simulink library "lib_IC_VSM"  (R2026a)
settings: Solver=VariableStepAuto
undefined symbols (not defined in the file): block_buses, block_DC_buses, block_DC_toM, block_idx, block_toM, buses_lf, DC, dparams, fb, fref, iC, inv2Hv, invL, iR, iTf, omegab, op_intconv_VSM
libraries: sl_discontinuities x1
(part 1 of 3)
settings Model: Creator=atomas  LastModifiedBy=atomas

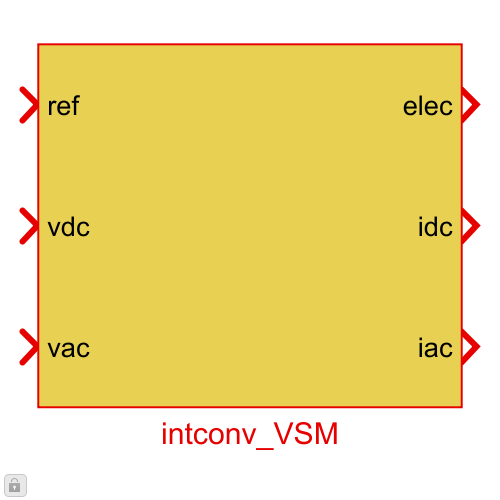
[thumbnail: Simulink's stored preview of the top-level diagram]
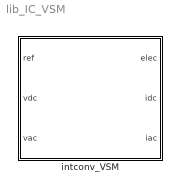
== system lib_IC_VSM ==
  intconv_VSM : Subsystem  mask(VCVSC){dynamic_VCC=Dynamic with P limitation, Lf=0.1, Rf=0.01, Rcf=1000000, Cfi=0.1, Kint=1, Tint=0.1, Bint=1, Kext=1, Bext=1, Text=0.1, Fi=1, Hv=3, Dv=0, Rv=0.05, nq=0.05, VI_L=0, VI_R=0, WOF_Tf=0, L_out=0.1, R_out=0.01, Tf=0.01, Kp_AC=0, Kd_AC=0, N_dc=100, Kp_theta=0, Kp_w=0, Ki_w=0, k_p_swing=1}
      mask prompts: dynamic_VCC "Dynamic behavior"; Lf "Filter inductance (pu)"; Rf "Filter resistance (pu)"; Rcf "Parallel resistance to C (pu)"; Cfi "Filter capacitance (pu)"; Fi "Current feedfordward gain"; Hv "Inertia"; Dv "Damping"; Rv "Droop Rv"; nq "Droop nq"; VI_L "Inductance (pu)"; VI_R "Resistance (pu)"; WOF_Tf "WOF time constant (s)"; L_out "Output inductance (p.u.)"; R_out "Output resistance (p.u.)"; Tf "Power filter time constant Tf (s):"; Kp_AC "DC-voltage proportional gain Kp_AC (pu):"; Kd_AC "DC-voltage derivative gain Kd_AC (pu*s):"; N_dc "DC-voltage derivative filter coefficient N_dc (rad/s):"; Kp_theta "ATM angle feed-forward gain Kp_theta (rad/pu):"; Kp_w "ATM frequency proportional gain Kp_w (pu/pu):"; Ki_w "ATM frequency integral gain Ki_w (pu/(pu*s)):"; k_p_swing "Swing equation DC-power coupling factor k_p_swing:"
      mask help: Grid-forming converter. VCC are the voltage and current controllers. Dynamic behavior includes the PI controllers, decoupling, current feedfordward and LC output filter. Static behavior consists of setting the reference voltage directly in the output. PC is the power controller including the droop control and low-pass filters for the power measurements.
      mask init:
      | [block_DC_buses, block_buses, block_DC_toM, block_toM, dparams, block_fref, block_idx, vcc_mode, use_wof_dc, use_kiw, use_Hv, inv2Hv] = mask_init_intconv_VSM(gcb, dynamic_VCC, Kd_AC, Ki_w, Hv);
      mask Help: web('Documentation/VCVSC.html')
      mask TypeOptions dynamic_VCC: Dynamic with limitation | Dynamic with P limitation | Dynamic | Static | Dynamic VC and static CC
      mask TypeOptions VI_L: VI/L
      mask TypeOptions VI_R: VI/R
      mask TypeOptions WOF_Tf: VI/Tf
      mask DialogControl Container8 Prompt: Parameters
      mask DialogControl VCC Prompt: VCC
      mask DialogControl PC Prompt: PC
      mask DialogControl VI Prompt: VI
      mask DialogControl Container9 Prompt: Others

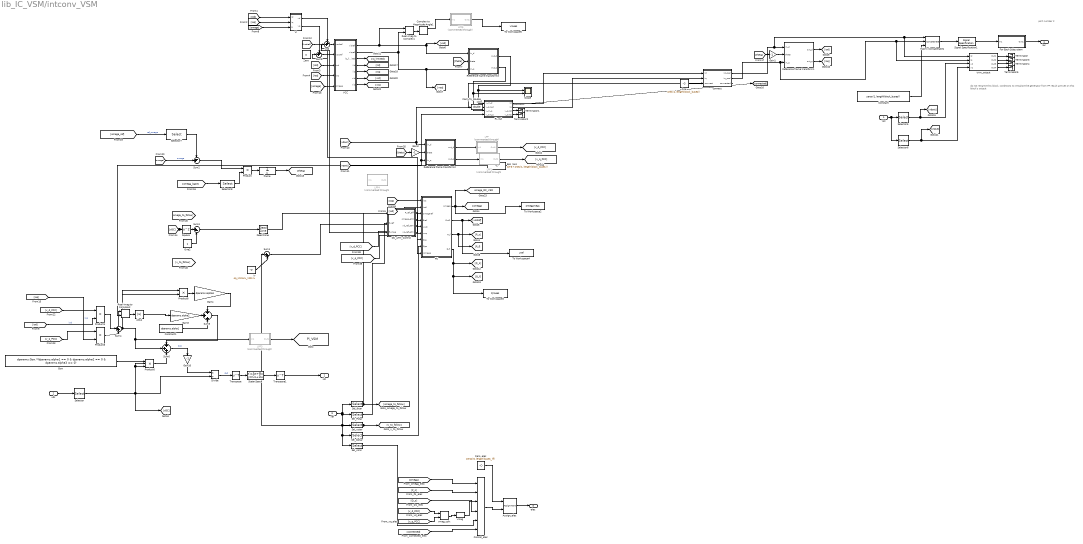
== system lib_IC_VSM/intconv_VSM ==
  note: do not rename this block, conditions to initialise the generator from PF result are set on this block's output
  note: port number 2
  vac : Inport
  vdc : Inport  Port=2
  ref : Inport  Port=3
  Abs4 : Abs  SaturateOnIntegerOverflow=off
  Assign_elec : Assignment  NumberOfDimensions=2  DiagnosticForDimensions=Warning  IndexOptions=Assign all,Index vector (dialog)  Indices=1,block_idx  OutputSizes=1
  Cast_To_Double_conn : DataTypeConversion  OutDataTypeStr=double
  Complex to Magnitude-Angle1 : ComplexToMagnitudeAngle
  Concat_elec : Concatenate  NumInputs=6  Mode=Multidimensional array
  Constant : Constant  Value=zeros(1, length(block_buses))  VectorParams1D=off
  Constant1 : Constant  Value=dparams.alpha1  VectorParams1D=off
  DC_ATM_Control : Subsystem
  Dead Zone : DeadZone  LowerValue=-0.2  UpperValue=0.2
  Divide : Product  Inputs=*/
  Eps_loss : Constant  Value=1e-6 * ones(1, length(block_buses))  VectorParams1D=off
  For Each Subsystem : Subsystem  TreatAsAtomicUnit=on
  Gain1 : Gain  Gain=-1
  Gain10 : Gain  Gain=-1
  Gain2 : Gain  Gain=-1
  Gain3 : Gain  Gain=dparams.alpha2
  Gain4 : Gain  Gain=dparams.alpha3
  Gsw : Constant  Value=dparams.Gsw.*(dparams.alpha1 == 0 & dparams.alpha2 == 0 & dparams.alpha3 == 0)  VectorParams1D=off
  LPF : Subsystem  Commented=through
  LPF1 : Subsystem  Commented=through
  LPF3 : Subsystem  Commented=through
  LPF4 : Subsystem  Commented=through
  LPF5 : Subsystem  Commented=through
  Matrix Concatenate1 : Concatenate  NumInputs=3  Mode=Multidimensional array
  One : Constant  Value=ones(1, length(block_buses))  VectorParams1D=off  OutDataTypeStr=Inherit: Inherit via back propagation
  One2 : Constant  OutDataTypeStr=Inherit: Inherit via back propagation
  PC : Subsystem  mask(PC_VCVSC){Tf=Tf, mp=0.01, nq=nq}
      mask prompts: Tf "Low-pass filter time constant (s)"; mp "Droop coefficient mp"; nq "Droop coefficient nq"
      mask help: Power controller of a grid-forming converter, including the droop control and low-pass filters for the power measurements.
      mask init:
      | [iTf, use_Tf] = mask_init_opt_filter(Tf);
  Product{,4..5,8} (4 alike) : Product
  Product6 : Product  Inputs=3
  RL out : Subsystem  Variant=on  mask{dynamic=Dynamic, R=dparams.Rf, L=dparams.Lf, fbase=50}
      mask prompts: dynamic "Dynamic behavior"; R "Series resistance (p.u.)"; L "Inductance (p.u.)"; fbase "Base frequency (Hz)"
      mask init:
      | [invL, omegab, rl_mode] = mask_init_RL(dynamic, L, fbase);
      mask TypeOptions dynamic: Static | Dynamic | Static omega
  Real-Imag to Complex1 : RealImagToComplex
  Real-Imag to Complex2 : RealImagToComplex
  Reference frame transform1 : Subsystem
  Reference frame transform2 : Subsystem
  Reference frame transform3 : Subsystem
  Scope : Scope  NumInputPorts=2
      settings: ActiveDisplayYMinimum=0.95813  ActiveDisplayYMaximum=1.0211
  Sel_Pstar : Selector  NumberOfDimensions=2  InputPortWidth=3  IndexOptions=Index vector (dialog),Index vector (dialog)  Indices=2,block_idx  OutputSizes=1
  Sel_Qstar : Selector  NumberOfDimensions=2  InputPortWidth=3  IndexOptions=Index vector (dialog),Index vector (dialog)  Indices=4,block_idx  OutputSizes=1
  Sel_conn : Selector  NumberOfDimensions=2  InputPortWidth=3  IndexOptions=Index vector (dialog),Index vector (dialog)  Indices=5,block_idx  OutputSizes=1
  Sel_fstar : Selector  NumberOfDimensions=2  InputPortWidth=3  IndexOptions=Index vector (dialog),Index vector (dialog)  Indices=1,block_idx  OutputSizes=1
  Sel_vstar : Selector  NumberOfDimensions=2  InputPortWidth=3  IndexOptions=Index vector (dialog),Index vector (dialog)  Indices=3,block_idx  OutputSizes=1
  Selector : Selector  InputPortWidth=DC.Nbuses  IndexOptions=Index vector (dialog)  Indices=block_DC_buses  OutputSizes=1
  Selector5 : Selector  NumberOfDimensions=2  InputPortWidth=3  IndexOptions=Index vector (dialog),Index vector (dialog)  Indices=1,block_buses  OutputSizes=1,1
  Selector6 : Selector  NumberOfDimensions=2  InputPortWidth=3  IndexOptions=Index vector (dialog),Index vector (dialog)  Indices=2,block_buses  OutputSizes=1,1
  Selector7 : Selector  InputPortWidth=length(fref.ref_units)  IndexOptions=Index vector (dialog)  Indices=block_fref  OutputSizes=1
  Selector8 : Selector  InputPortWidth=length(fref.ref_units)  IndexOptions=Index vector (dialog)  Indices=block_fref  OutputSizes=1
  Signal Specification1 : SignalSpecification  Dimensions=[3 length(block_buses)]
  Square : Math  Operator=square
  State-Space : StateSpace  A=[]  B=[]  C=[]  D=block_DC_toM  InitialCondition=0  ParameterTunability=Optimized
  Sum1 : Sum  Inputs=|++
  Sum2 : Sum  Inputs=-+|
  Sum3 : Sum  Inputs=|+-
  Sum4 : Sum  Inputs=|++
  Sum5 : Sum  Inputs=+|+|+
  Sum6 : Sum  Inputs=+|+|+
  Sum8 : Sum  Inputs=++|
  Terminator{,1..5} (6 alike) : Terminator
  To Workspace2 : ToWorkspace  VariableName=omegameas  SaveFormat=Timeseries  SampleTime=-1
  To Workspace3 : ToWorkspace  VariableName=Qmeas  SaveFormat=Timeseries  SampleTime=-1
  To Workspace4 : ToWorkspace  VariableName=vref  SaveFormat=Timeseries  SampleTime=-1
  To Workspace5 : ToWorkspace  VariableName=vmeas  SaveFormat=Timeseries  SampleTime=-1
  Transpose : Math  Operator=transpose
  Transpose1 : Math  Operator=transpose
  VCC : Subsystem  Variant=on
  VI : Subsystem  mask{L=VI_L, R=VI_R, Tf=WOF_Tf}
      mask prompts: L "Inductance (pu)"; R "Resistance (pu)"; Tf "WOF time constant (s)"
      mask init:
      | [iTf, use_Tf] = mask_init_opt_filter(Tf);
  Zero : Constant  Value=0  OutDataTypeStr=Inherit: Inherit via back propagation
  Zero_elec : Constant  Value=zeros(6, length(buses_lf))
  connect : Subsystem
  frame : Integrator  InitialCondition=op_intconv_VSM.frame  IgnoreLimit=on
  iv : Constant  Value=op_intconv_VSM.iv  VectorParams1D=off
  trim_output : Subsystem
  vmag : ComplexToMagnitudeAngle  Output=Magnitude
  vmag_cplx : RealImagToComplex
  vod : Sum  Inputs=++|
  iac : Outport
  idc : Outport  Port=2
  elec : Outport  Port=3
  tag scope: Pi_VSM=global, omega_DC_VSM=global
  wires:
  Sum8/1 -> VCC/2(voqref)
  vod/1 -> VCC/1(vodref)
  [omega] -> VI/3(omega)
  [ioq] -> VI/2(iq)
  [iod] -> VI/1(id)
  Gain2/1 -> Reference frame transform2/2(theta)
  [theta] -> Gain2/1
  PC/4(Q_f) -> [Q_s], To Workspace3/1, [Q_f]
  PC/3(P_f) -> [P_s], [P_f]
  [omega] -> Sum2/2  "omega"
  [omega_ref] -> Selector7/1  "ref_omega"
  RL out/1(id) -> connect/1(id)
  [theta] -> Gain1/1
  Gain1/1 -> Reference frame transform1/2(theta)
  [ioq] -> VCC/4(ioq)
  [iod] -> VCC/3(iod)
  [omega] -> VCC/5(omega)
  [theta] -> Reference frame transform3/2(theta)
  PC/1(omega) -> To Workspace2/1, [omega_DC_VSM], [omega]
  PC/2(Out2) -> To Workspace4/1, [vodref]
  [iod] -> PC/2(iodi)
  [ioq] -> PC/1(ioq)
  Reference frame transform1/2(out_q) -> [ioq]
  Reference frame transform3/1(out_d) -> RL out/1(v_in_d), Scope/1
  Reference frame transform3/2(out_q) -> RL out/3(v_in_q), Scope/2
  RL out/2(iq) -> connect/2(iq)
  Reference frame transform1/1(out_d) -> [iod]
  VI/1(vd) -> vod/1
  VI/2(vq) -> Sum8/1
  connect/1(id_real) -> trim_output/1(id), Matrix Concatenate1/1, Reference frame transform1/1(in_d)
  connect/2(iq_real) -> trim_output/2(iq), Matrix Concatenate1/2, Reference frame transform1/3(in_q)
  RL out/3(v_outd) -> Terminator1/1
  RL out/4(v_outq) -> Terminator2/1
  Reference frame transform2/1(out_d) -> LPF/1(In1)
  Reference frame transform2/2(out_q) -> LPF1/1(In1)
  [vqout] -> Reference frame transform2/3(in_q), RL out/4(v_out_q)
  LPF/1(Out1) -> [v_d_PCC]
  LPF1/1(Out1) -> [v_q_PCC]
  [vdout] -> RL out/2(v_out_d), Reference frame transform2/1(in_d)
  Matrix Concatenate1/1 -> Signal Specification1/1
  Constant/1 -> Matrix Concatenate1/3
  For Each Subsystem/1(Out1) -> iac/1
  Signal Specification1/1 -> For Each Subsystem/1(In1)
  [v_d_PCC] -> PC/5(vodi)
  [v_q_PCC] -> PC/6(voq)
  trim_output/1(Out1) -> Terminator/1
  trim_output/2(Out2) -> Terminator3/1
  trim_output/3(Out3) -> Terminator4/1
  trim_output/4(Out4) -> Terminator5/1
  vac/1 -> Selector6/1, Selector5/1
  Selector6/1 -> [vqout], trim_output/4(vq)
  Selector5/1 -> [vdout], trim_output/3(vd)
  VCC/1(vidref) -> Real-Imag to Complex1/1, [vod], Reference frame transform3/1(in_d)
  VCC/2(viqref) -> [voq], Reference frame transform3/3(in_q), Real-Imag to Complex1/2
  One/1 -> connect/3(connect)
  Sum1/1 -> PC/4(Eref)
  vdc/1 -> Selector/1
  Transpose/1 -> State-Space/1
  Divide/1 -> Transpose/1  "iDC"
  Abs4/1 -> Gain3/1
  Transpose1/1 -> idc/1
  Product5/1 -> Sum4/2
  Product6/1 -> Sum6/3
  Sum4/1 -> LPF3/1(In1), Sum6/2, Product8/1, Product8/2, Real-Imag to Complex2/1
  Sum5/1 -> Sum6/1
  State-Space/1 -> Transpose1/1
  Gain4/1 -> Sum5/1
  Gsw/1 -> Product6/1
  Real-Imag to Complex2/1 -> Abs4/1
  Constant1/1 -> Sum5/3
  Product4/1 -> Sum4/1
  Sum6/1 -> Gain10/1  "Pdc"
  Gain3/1 -> Sum5/2
  Gain10/1 -> Divide/1
  Product8/1 -> Gain4/1
  [v_q_PCC] -> Product5/1
  Selector/1 -> Product6/3, Product6/2, [vDC], Divide/2
  [ioq] -> Product5/2  "ioq"
  [v_d_PCC] -> Product4/1
  [iod] -> Product4/2  "iod"
  Product/1 -> frame/1
  VCC/3(iq_limited) -> [iq_limited]
  VCC/4(iid) -> [iid]
  VCC/5(iiq) -> [iiq]
  VCC/6(vid) -> [vid]
  VCC/7(viq) -> [viq]
  [vDC] -> Square/1, DC_ATM_Control/1(v_dc)
  Square/1 -> Sum3/1
  One2/1 -> Sum3/2
  frame/1 -> [theta]
  Sum3/1 -> Dead Zone/1
  LPF3/1(Out1) -> [Pi_VSM]
  Real-Imag to Complex1/1 -> Complex to Magnitude-Angle1/1
  Complex to Magnitude-Angle1/1 -> LPF5/1(In1)
  LPF5/1(Out1) -> To Workspace5/1
  Selector8/1 -> Product/2
  [omega_base] -> Selector8/1
  Sum2/1 -> Product/1
  Selector7/1 -> Sum2/1
  ref/1 -> Sel_Qstar/1, Sel_conn/1, Sel_vstar/1, Sel_Pstar/1, Sel_fstar/1
  Sel_fstar/1 -> [omega_to_follow], PC/3(omegaref)
  Sel_vstar/1 -> [v_to_follow], Sum1/1
  Sel_Qstar/1 -> PC/8(Qsp)
  [v_d_PCC] -> vmag_cplx/1
  [v_q_PCC] -> vmag_cplx/2
  vmag_cplx/1 -> vmag/1
  [omega] -> Concat_elec/1
  [P_s] -> Concat_elec/2
  vmag/1 -> Concat_elec/3
  [Q_s] -> Concat_elec/4
  Sel_conn/1 -> Concat_elec/5
  [connected] -> Concat_elec/6
  Zero_elec/1 -> Assign_elec/1
  Concat_elec/1 -> Assign_elec/2
  Assign_elec/1 -> elec/1
  Sel_Pstar/1 -> DC_ATM_Control/2(P_ref)
  [vodref] -> DC_ATM_Control/3(E_mag)
  DC_ATM_Control/1(P_ref_eff) -> PC/7(Psp)
  DC_ATM_Control/2(omega_atm) -> PC/9(iomega)
  DC_ATM_Control/3(vd_ref_atm) -> vod/2
  DC_ATM_Control/4(vq_ref_atm) -> Sum8/2
  iv/1 -> Sum1/2
  Eps_loss/1 -> Real-Imag to Complex2/2
  connect/3(connected) -> Cast_To_Double_conn/1
  Cast_To_Double_conn/1 -> [connected]

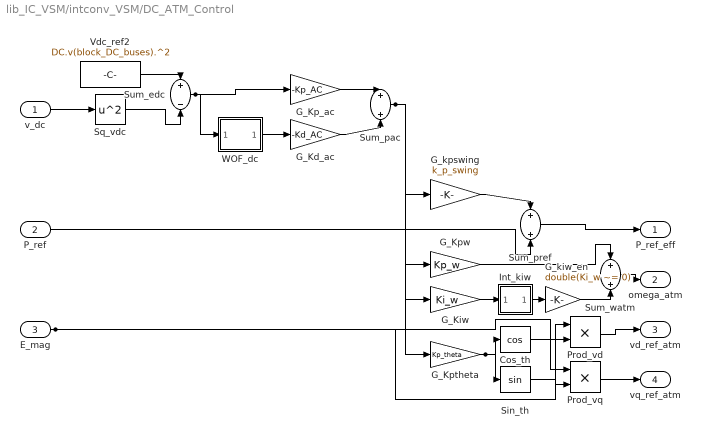
== system lib_IC_VSM/intconv_VSM/DC_ATM_Control ==
  v_dc : Inport
  P_ref : Inport  Port=2
  E_mag : Inport  Port=3
  Cos_th : Trigonometry  Operator=cos
  G_Kd_ac : Gain  Gain=-Kd_AC
  G_Kiw : Gain  Gain=Ki_w
  G_Kp_ac : Gain  Gain=-Kp_AC
  G_Kptheta : Gain  Gain=Kp_theta
  G_Kpw : Gain  Gain=Kp_w
  G_kiw_en : Gain  Gain=double(Ki_w ~= 0)
  G_kpswing : Gain  Gain=k_p_swing
  Int_kiw : Subsystem  Variant=on
  Prod_vd : Product  Inputs=**
  Prod_vq : Product  Inputs=**
  Sin_th : Trigonometry
  Sq_vdc : Math  Operator=square
  Sum_edc : Sum  Inputs=+-
  Sum_pac : Sum
  Sum_pref : Sum
  Sum_watm : Sum
  Vdc_ref2 : Constant  Value=DC.v(block_DC_buses).^2
  WOF_dc : Subsystem  Variant=on
  P_ref_eff : Outport
  omega_atm : Outport  Port=2
  vd_ref_atm : Outport  Port=3
  vq_ref_atm : Outport  Port=4
  wires:
  Int_kiw/1(Out1) -> G_kiw_en/1
  G_Kiw/1 -> Int_kiw/1(In1)
  WOF_dc/1(Out1) -> G_Kd_ac/1
  Sum_edc/1 -> WOF_dc/1(In1), G_Kp_ac/1
  v_dc/1 -> Sq_vdc/1
  Vdc_ref2/1 -> Sum_edc/1
  Sq_vdc/1 -> Sum_edc/2
  G_Kp_ac/1 -> Sum_pac/1
  G_Kd_ac/1 -> Sum_pac/2
  Sum_pac/1 -> G_kpswing/1, G_Kpw/1, G_Kiw/1, G_Kptheta/1
  G_kpswing/1 -> Sum_pref/1
  P_ref/1 -> Sum_pref/2
  Sum_pref/1 -> P_ref_eff/1
  G_Kpw/1 -> Sum_watm/1
  G_kiw_en/1 -> Sum_watm/2
  Sum_watm/1 -> omega_atm/1
  G_Kptheta/1 -> Cos_th/1, Sin_th/1
  E_mag/1 -> Prod_vd/1, Prod_vq/1
  Cos_th/1 -> Prod_vd/2
  Sin_th/1 -> Prod_vq/2
  Prod_vd/1 -> vd_ref_atm/1
  Prod_vq/1 -> vq_ref_atm/1

== system lib_IC_VSM/intconv_VSM/For Each Subsystem ==
  In1 : Inport  Partition=on  PartitionDimension=1  PartitionWidth=1  PartitionOffset=0
  For Each : ForEach  DisableCoverage=on
  State-Space : StateSpace  A=[]  B=[]  C=[]  D=block_toM  InitialCondition=0  ParameterTunability=Optimized
  Transpose : Math  Operator=transpose
  Transpose1 : Math  Operator=transpose
  Out1 : Outport  ConcatenationDimension=1
  wires:
  State-Space/1 -> Transpose1/1
  Transpose/1 -> State-Space/1
  Transpose1/1 -> Out1/1
  In1/1 -> Transpose/1

== system lib_IC_VSM/intconv_VSM/LPF ==
  In1 : Inport
  Gain : Gain  Gain=1e2
  I : Integrator  InitialCondition=op_intconv_VSM.LPF_I
  Sum4 : Sum  Inputs=|+-
  Out1 : Outport
  wires:
  Gain/1 -> I/1
  Sum4/1 -> Gain/1
  In1/1 -> Sum4/1
  I/1 -> Out1/1, Sum4/2

== system lib_IC_VSM/intconv_VSM/LPF1 ==
  In1 : Inport
  Gain : Gain  Gain=1e2
  I : Integrator  InitialCondition=op_intconv_VSM.LPF1_I
  Sum4 : Sum  Inputs=|+-
  Out1 : Outport
  wires:
  I/1 -> Sum4/2, Out1/1
  In1/1 -> Sum4/1
  Sum4/1 -> Gain/1
  Gain/1 -> I/1

== system lib_IC_VSM/intconv_VSM/LPF3 ==
  In1 : Inport
  Gain : Gain  Gain=1000
  I : Integrator  InitialCondition=op_intconv_VSM.LPF3_I
  Sum4 : Sum  Inputs=|+-
  Out1 : Outport
  wires:
  Gain/1 -> I/1
  Sum4/1 -> Gain/1
  In1/1 -> Sum4/1
  I/1 -> Out1/1, Sum4/2

== system lib_IC_VSM/intconv_VSM/LPF4 ==
  In1 : Inport
  Gain : Gain  Gain=1e2
  I : Integrator  InitialCondition=op_intconv_VSM.LPF4_I
  Sum4 : Sum  Inputs=|+-
  Out1 : Outport
  wires:
  Gain/1 -> I/1
  Sum4/1 -> Gain/1
  In1/1 -> Sum4/1
  I/1 -> Out1/1, Sum4/2

== system lib_IC_VSM/intconv_VSM/LPF5 ==
  In1 : Inport
  Gain : Gain  Gain=1e4
  I : Integrator  InitialConditionSource=external  InitialCondition=op_intconv_VSM.LPF5_I
  Sum4 : Sum  Inputs=|+-
  Out1 : Outport
  wires:
  Gain/1 -> I/1
  Sum4/1 -> Gain/1
  In1/1 -> I/2, Sum4/1
  I/1 -> Out1/1, Sum4/2

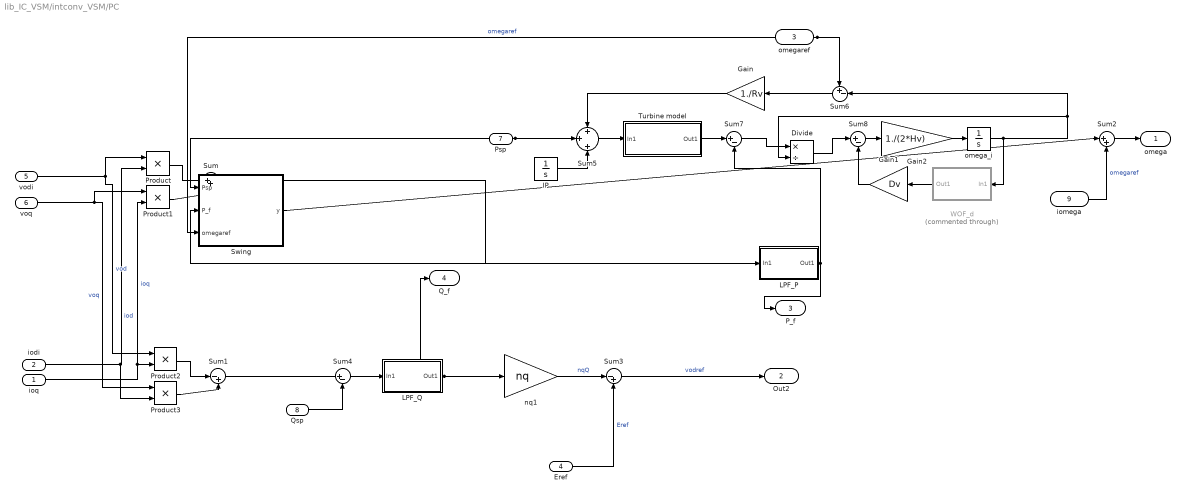
== system lib_IC_VSM/intconv_VSM/PC ==
  ioq : Inport
  iodi : Inport  Port=2
  omegaref : Inport  Port=3
  Eref : Inport  Port=4
  vodi : Inport  Port=5
  voq : Inport  Port=6
  Psp : Inport  Port=7
  Qsp : Inport  Port=8
  iomega : Inport  Port=9
  Divide : Product  Inputs=*/
  Gain : Gain  Gain=1./Rv
  Gain1 : Gain  Gain=Dv
  Gain2 : Gain  Gain=1./(2*Hv)
  IP : Integrator  InitialCondition=op_intconv_VSM.PC_IP
  LPF_P : Subsystem  Variant=on
  LPF_Q : Subsystem  Variant=on
  Product{,1..3} (4 alike) : Product
  Sum : Sum  Inputs=|++
  Sum1 : Sum  Inputs=|-+
  Sum2 : Sum  Inputs=|++
  Sum3 : Sum  Inputs=|-+
  Sum4 : Sum  Inputs=|+-
  Sum5 : Sum  Inputs=+|+|+
  Sum6 : Sum  Inputs=+-|
  Sum7 : Sum  Inputs=|+-
  Sum8 : Sum  Inputs=|+-
  Swing : Subsystem  Variant=on
  Turbine model : Subsystem
  WOF_d : Subsystem  Commented=through
  nq1 : Gain  Gain=nq
  omega_i : Integrator  InitialCondition=op_intconv_VSM.PC_omega_i
  omega : Outport
  Out2 : Outport  Port=2
  P_f : Outport  Port=3
  Q_f : Outport  Port=4
  wires:
  LPF_P/1(Out1) -> Sum7/2, P_f/1, Swing/2(P_f)
  Sum/1 -> LPF_P/1(In1)
  vodi/1 -> Product2/1, Product/1  "vod"
  Product/1 -> Sum/1
  Product1/1 -> Sum/2
  Product2/1 -> Sum1/1
  Product3/1 -> Sum1/2
  nq1/1 -> Sum3/1  "nqQ"
  Eref/1 -> Sum3/2  "Eref"
  voq/1 -> Product1/1, Product3/1  "voq"
  iodi/1 -> Product3/2, Product/2  "iod"
  ioq/1 -> Product2/2, Product1/2  "ioq"
  Qsp/1 -> Sum4/2
  Sum3/1 -> Out2/1  "vodref"
  Gain2/1 -> omega_i/1
  Sum6/1 -> Gain/1
  omega_i/1 -> WOF_d/1(In1), Sum6/2, Divide/2
  Gain/1 -> Sum5/1
  WOF_d/1(Out1) -> Gain1/1
  Turbine model/1(Out1) -> Sum7/1
  Gain1/1 -> Sum8/2
  Divide/1 -> Sum8/1
  Psp/1 -> Sum5/2, Swing/1(Psp)
  Sum5/1 -> Turbine model/1(In1)
  Sum7/1 -> Divide/1
  Sum8/1 -> Gain2/1
  IP/1 -> Sum5/3
  omegaref/1 -> Sum6/1, Swing/3(omegaref)  "omegaref"
  Sum2/1 -> omega/1
  iomega/1 -> Sum2/2  "omegaref"
  Sum1/1 -> LPF_Q/1(In1)
  LPF_Q/1(Out1) -> Q_f/1, Sum4/1
  Sum4/1 -> nq1/1
  Swing/1(y) -> Sum2/1

== system lib_IC_VSM/intconv_VSM/RL out ==
  note: 1) Add Subsystem or Model blocks as valid variant choices.
      | 2) You cannot connect blocks at this level. At simulation, connectivity is automatically
      | determined, based on the active variant and port name matching.
  v_in_d : Inport
  v_out_d : Inport  Port=2
  v_in_q : Inport  Port=3
  v_out_q : Inport  Port=4
  dynamic : Subsystem  VariantControl=rl_mode == 1
  static : Subsystem  VariantControl=rl_mode == 2
  static_omega : Subsystem  VariantControl=(default)
  id : Outport
  iq : Outport  Port=2
  v_outd : Outport  Port=3
  v_outq : Outport  Port=4

== system lib_IC_VSM/intconv_VSM/Reference frame transform1 ==
  in_d : Inport
  theta : Inport  Port=2
  in_q : Inport  Port=3
  Complex to Real-Imag : ComplexToRealImag
  Cos : Trigonometry  SCDEnableBlockLinearizationSpecification=on  Operator=cos
  Product : Product
  Real-Imag to Complex : RealImagToComplex
  Real-Imag to Complex1 : RealImagToComplex
  Sin : Trigonometry  SCDEnableBlockLinearizationSpecification=on
  out_d : Outport
  out_q : Outport  Port=2
  wires:
  Complex to Real-Imag/2 -> out_q/1
  Real-Imag to Complex1/1 -> Product/1
  Real-Imag to Complex/1 -> Product/2
  Product/1 -> Complex to Real-Imag/1
  theta/1 -> Sin/1, Cos/1
  Cos/1 -> Real-Imag to Complex1/1
  Sin/1 -> Real-Imag to Complex1/2
  Complex to Real-Imag/1 -> out_d/1
  in_q/1 -> Real-Imag to Complex/2
  in_d/1 -> Real-Imag to Complex/1

== system lib_IC_VSM/intconv_VSM/Reference frame transform2 ==
  in_d : Inport
  theta : Inport  Port=2
  in_q : Inport  Port=3
  Complex to Real-Imag : ComplexToRealImag
  Cos : Trigonometry  SCDEnableBlockLinearizationSpecification=on  Operator=cos
  Product : Product
  Real-Imag to Complex : RealImagToComplex
  Real-Imag to Complex1 : RealImagToComplex
  Sin : Trigonometry  SCDEnableBlockLinearizationSpecification=on
  out_d : Outport
  out_q : Outport  Port=2
  wires:
  in_d/1 -> Real-Imag to Complex/1
  in_q/1 -> Real-Imag to Complex/2
  Complex to Real-Imag/1 -> out_d/1
  Sin/1 -> Real-Imag to Complex1/2
  Cos/1 -> Real-Imag to Complex1/1
  theta/1 -> Cos/1, Sin/1
  Product/1 -> Complex to Real-Imag/1
  Real-Imag to Complex/1 -> Product/2
  Real-Imag to Complex1/1 -> Product/1
  Complex to Real-Imag/2 -> out_q/1

== system lib_IC_VSM/intconv_VSM/Reference frame transform3 ==
  in_d : Inport
  theta : Inport  Port=2
  in_q : Inport  Port=3
  Complex to Real-Imag : ComplexToRealImag
  Cos : Trigonometry  SCDEnableBlockLinearizationSpecification=on  Operator=cos
  Product : Product
  Real-Imag to Complex : RealImagToComplex
  Real-Imag to Complex1 : RealImagToComplex
  Sin : Trigonometry  SCDEnableBlockLinearizationSpecification=on
  out_d : Outport
  out_q : Outport  Port=2
  wires:
  Complex to Real-Imag/2 -> out_q/1
  Real-Imag to Complex1/1 -> Product/1
  Real-Imag to Complex/1 -> Product/2
  Product/1 -> Complex to Real-Imag/1
  theta/1 -> Cos/1, Sin/1
  Cos/1 -> Real-Imag to Complex1/1
  Sin/1 -> Real-Imag to Complex1/2
  Complex to Real-Imag/1 -> out_d/1
  in_q/1 -> Real-Imag to Complex/2
  in_d/1 -> Real-Imag to Complex/1

== system lib_IC_VSM/intconv_VSM/VCC ==
  note: 1) Add Subsystem or Model blocks as valid variant choices.
      | 2) You cannot connect blocks at this level. At simulation, connectivity is automatically
      | determined, based on the active variant and port name matching.
  vodref : Inport
  voqref : Inport  Port=2
  iod : Inport  Port=3
  ioq : Inport  Port=4
  omega : Inport  Port=5
  dynamic : Subsystem  VariantControl=vcc_mode == 1
  dynamic_VC : Subsystem  VariantControl=vcc_mode == 3
  dynamic_limiting : Subsystem  VariantControl=vcc_mode == 2
  dynamic_limiting_P : Subsystem  VariantControl=vcc_mode == 4
  static : Subsystem  VariantControl=(default)
  vidref : Outport
  viqref : Outport  Port=2
  iq_limited : Outport  Port=3
  iid : Outport  Port=4
  iiq : Outport  Port=5
  vid : Outport  Port=6
  viq : Outport  Port=7

== system lib_IC_VSM/intconv_VSM/VI ==
  id : Inport
  iq : Inport  Port=2
  omega : Inport  Port=3
  Gain : Gain  Gain=L
  Gain1 : Gain  Gain=R
  Gain2 : Gain  Gain=L
  Gain3 : Gain  Gain=R
  Product : Product
  Product1 : Product
  Sum : Sum  Inputs=-+|
  Sum1 : Sum  Inputs=|--
  WOF_d : Subsystem  Variant=on
  WOF_q : Subsystem  Variant=on
  vd : Outport
  vq : Outport  Port=2
  wires:
  WOF_q/1(Out1) -> Gain/1, Gain3/1
  iq/1 -> WOF_q/1(In1)
  WOF_d/1(Out1) -> Gain1/1, Gain2/1
  id/1 -> WOF_d/1(In1)
  Sum1/1 -> vq/1
  Sum/1 -> vd/1
  Gain3/1 -> Sum1/2
  Gain1/1 -> Sum/1
  Product1/1 -> Sum1/1
  Gain2/1 -> Product1/2
  Product/1 -> Sum/2
  omega/1 -> Product1/1, Product/2
  Gain/1 -> Product/1

== system lib_IC_VSM/intconv_VSM/connect ==
  id : Inport
  iq : Inport  Port=2
  connect : Inport  Port=3
  Switch : Switch  Criteria=u2 > Threshold  ZeroCross=off  SaturateOnIntegerOverflow=off  InputSameDT=off
  Switch1 : Switch  Criteria=u2 > Threshold  ZeroCross=off  SaturateOnIntegerOverflow=off  InputSameDT=off
  Zero1 : Constant  Value=0  VectorParams1D=off  OutDataTypeStr=Inherit: Inherit via back propagation
  Zero2 : Constant  Value=0  VectorParams1D=off  OutDataTypeStr=Inherit: Inherit via back propagation
  id_real : Outport
  iq_real : Outport  Port=2
  connected : Outport  Port=3  OutDataTypeStr=boolean
  wires:
  Switch/1 -> id_real/1
  Zero1/1 -> Switch/3
  id/1 -> Switch/1
  connect/1 -> connected/1, Switch1/2, Switch/2
  Switch1/1 -> iq_real/1
  iq/1 -> Switch1/1
  Zero2/1 -> Switch1/3

== system lib_IC_VSM/intconv_VSM/trim_output ==
  id : Inport
  iq : Inport  Port=2
  vd : Inport  Port=3
  vq : Inport  Port=4
  Out1 : Outport
  Out2 : Outport  Port=2
  Out3 : Outport  Port=3
  Out4 : Outport  Port=4
  wires:
  id/1 -> Out1/1
  vq/1 -> Out4/1
  vd/1 -> Out3/1
  iq/1 -> Out2/1

== system lib_IC_VSM/intconv_VSM/DC_ATM_Control/Int_kiw ==
  note: 1) Add Subsystem or Model blocks as valid variant choices.
      | 2) You cannot connect blocks at this level. At simulation, connectivity is automatically
      | determined, based on the active variant and port name matching.
  In1 : Inport
  Active : Subsystem  VariantControl=use_kiw == 1
  Bypass : Subsystem  VariantControl=(default)
  Out1 : Outport

== system lib_IC_VSM/intconv_VSM/DC_ATM_Control/WOF_dc ==
  note: 1) Add Subsystem or Model blocks as valid variant choices.
      | 2) You cannot connect blocks at this level. At simulation, connectivity is automatically
      | determined, based on the active variant and port name matching.
  In1 : Inport
  Active : Subsystem  VariantControl=use_wof_dc == 1
  Bypass : Subsystem  VariantControl=(default)
  Out1 : Outport

== system lib_IC_VSM/intconv_VSM/PC/LPF_P ==
  note: 1) Add Subsystem or Model blocks as valid variant choices.
      | 2) You cannot connect blocks at this level. At simulation, connectivity is automatically
      | determined, based on the active variant and port name matching.
  In1 : Inport
  Active : Subsystem  VariantControl=use_Tf == 1
  Bypass : Subsystem  VariantControl=(default)
  Out1 : Outport

== system lib_IC_VSM/intconv_VSM/PC/LPF_Q ==
  note: 1) Add Subsystem or Model blocks as valid variant choices.
      | 2) You cannot connect blocks at this level. At simulation, connectivity is automatically
      | determined, based on the active variant and port name matching.
  In1 : Inport
  Active : Subsystem  VariantControl=use_Tf == 1
  Bypass : Subsystem  VariantControl=(default)
  Out1 : Outport

== system lib_IC_VSM/intconv_VSM/PC/Swing ==
  note: 1) Add Subsystem or Model blocks as valid variant choices.
      | 2) You cannot connect blocks at this level. At simulation, connectivity is automatically
      | determined, based on the active variant and port name matching.
  Psp : Inport
  P_f : Inport  Port=2
  omegaref : Inport  Port=3
  Active : Subsystem  VariantControl=use_Hv == 1
  Droop : Subsystem  VariantControl=(default)
  y : Outport

== system lib_IC_VSM/intconv_VSM/PC/Turbine model ==
  In1 : Inport
  Out1 : Outport
  wires:
  In1/1 -> Out1/1

== system lib_IC_VSM/intconv_VSM/PC/WOF_d ==
  In1 : Inport
  Gain : Gain  Gain=10
  Gain1 : Gain  Gain=10
  I : Integrator  InitialConditionSource=external  InitialCondition=op_intconv_VSM.PC_WOF_d_I
  Sum : Sum  Inputs=+-|
  Sum4 : Sum  Inputs=|+-
  Out1 : Outport
  wires:
  Gain/1 -> I/1
  Sum4/1 -> Gain/1
  In1/1 -> I/2, Sum/1, Sum4/1
  I/1 -> Sum/2, Sum4/2
  Sum/1 -> Gain1/1
  Gain1/1 -> Out1/1

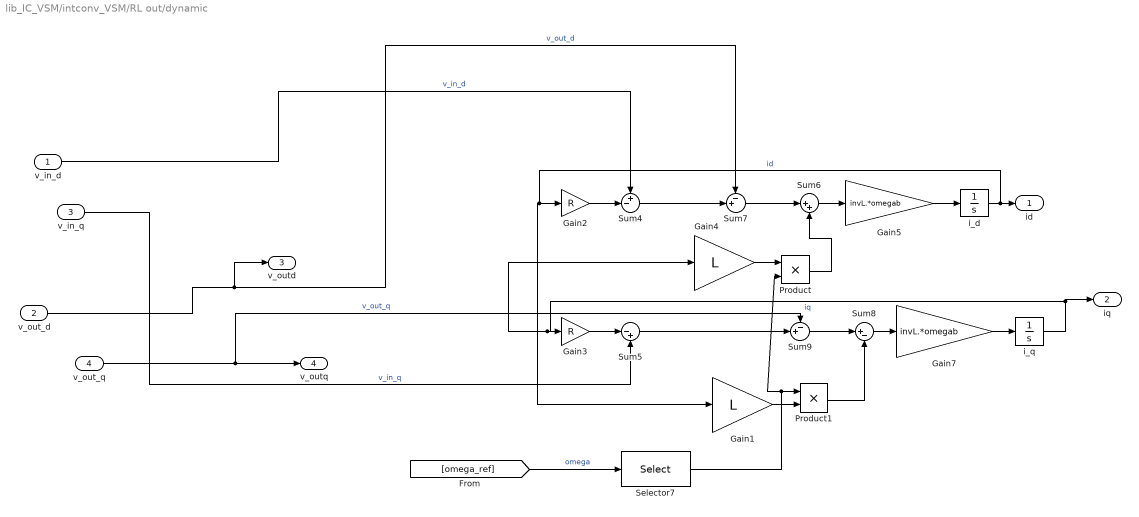
== system lib_IC_VSM/intconv_VSM/RL out/dynamic ==
  v_in_d : Inport
  v_out_d : Inport  Port=2
  v_in_q : Inport  Port=3
  v_out_q : Inport  Port=4
  Gain1 : Gain  Gain=L
  Gain2 : Gain  Gain=R
  Gain3 : Gain  Gain=R
  Gain4 : Gain  Gain=L
  Gain5 : Gain  Gain=invL.*omegab
  Gain7 : Gain  Gain=invL.*omegab
  Product : Product
  Product1 : Product
  Selector7 : Selector  InputPortWidth=length(fref.ref_units)  IndexOptions=Index vector (dialog)  Indices=block_fref  OutputSizes=1
  Sum4 : Sum  Inputs=+-|
  Sum5 : Sum  Inputs=|-+
  Sum6 : Sum  Inputs=|++
  Sum7 : Sum  Inputs=-+|
  Sum8 : Sum  Inputs=|+-
  Sum9 : Sum  Inputs=-+|
  i_d : Integrator  InitialCondition=op_intconv_VSM.RL_out_dynamic_i_d
  i_q : Integrator  InitialCondition=op_intconv_VSM.RL_out_dynamic_i_q
  id : Outport
  iq : Outport  Port=2
  v_outd : Outport  Port=3
  v_outq : Outport  Port=4
  wires:
  v_out_q/1 -> v_outq/1, Sum9/1  "v_out_q"
  v_out_d/1 -> v_outd/1, Sum7/1  "v_out_d"
  Sum9/1 -> Sum8/1
  Gain1/1 -> Product1/2
  i_q/1 -> iq/1, Gain4/1, Gain3/1  "iq"
  Gain7/1 -> i_q/1
  Sum5/1 -> Sum9/2
  Gain3/1 -> Sum5/1
  Sum7/1 -> Sum6/1
  Gain4/1 -> Product/1
  Product1/1 -> Sum8/2
  Sum4/1 -> Sum7/2
  Sum8/1 -> Gain7/1
  Product/1 -> Sum6/2
  Gain5/1 -> i_d/1
  [omega_ref] -> Selector7/1  "omega"
  Sum6/1 -> Gain5/1
  i_d/1 -> id/1, Gain1/1, Gain2/1  "id"
  Gain2/1 -> Sum4/2
  v_in_d/1 -> Sum4/1  "v_in_d"
  v_in_q/1 -> Sum5/2  "v_in_q"
  Selector7/1 -> Product/2, Product1/1

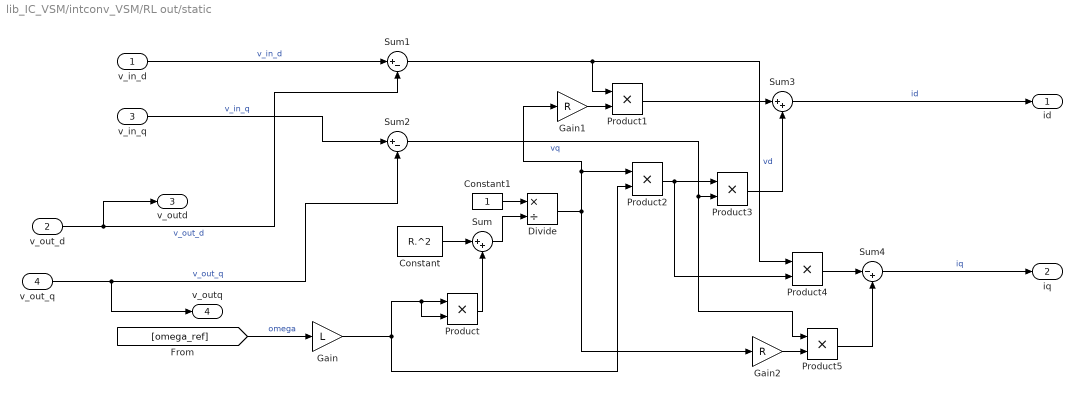
== system lib_IC_VSM/intconv_VSM/RL out/static ==
  v_in_d : Inport
  v_out_d : Inport  Port=2
  v_in_q : Inport  Port=3
  v_out_q : Inport  Port=4
  Constant : Constant  Value=R.^2
  Constant1 : Constant
  Divide : Product  Inputs=*/
  Gain : Gain  Gain=L
  Gain1 : Gain  Gain=R
  Gain2 : Gain  Gain=R
  Product{,1..5} (6 alike) : Product
  Sum : Sum  Inputs=|++
  Sum1 : Sum  Inputs=|+-
  Sum2 : Sum  Inputs=|+-
  Sum3 : Sum  Inputs=|++
  Sum4 : Sum  Inputs=|-+
  id : Outport
  iq : Outport  Port=2
  v_outd : Outport  Port=3
  v_outq : Outport  Port=4
  wires:
  [omega_ref] -> Gain/1  "omega"
  v_in_d/1 -> Sum1/1  "v_in_d"
  v_out_q/1 -> v_outq/1, Sum2/2  "v_out_q"
  Sum4/1 -> iq/1  "iq"
  Sum3/1 -> id/1  "id"
  Gain1/1 -> Product1/2
  Product2/1 -> Product4/2, Product3/1
  Product4/1 -> Sum4/1
  Divide/1 -> Gain2/1, Gain1/1, Product2/1
  Sum1/1 -> Product1/1, Product4/1  "vd"
  Product3/1 -> Sum3/2
  Constant1/1 -> Divide/1
  Gain/1 -> Product/2, Product/1, Product2/2
  Sum2/1 -> Product5/1, Product3/2  "vq"
  Constant/1 -> Sum/1
  Product5/1 -> Sum4/2
  Product1/1 -> Sum3/1
  Product/1 -> Sum/2
  Gain2/1 -> Product5/2
  Sum/1 -> Divide/2
  v_out_d/1 -> v_outd/1, Sum1/2  "v_out_d"
  v_in_q/1 -> Sum2/1  "v_in_q"

== system lib_IC_VSM/intconv_VSM/RL out/static_omega ==
  v_in_d : Inport
  v_out_d : Inport  Port=2
  v_in_q : Inport  Port=3
  v_out_q : Inport  Port=4
  Gain : Gain  Gain=1./(R.^2+L.^2)
  Gain2 : Gain  Gain=1./(R.^2+L.^2)
  Gain3 : Gain  Gain=R
  Gain4 : Gain  Gain=L
  Gain5 : Gain  Gain=L
  Gain6 : Gain  Gain=R
  Sum : Sum  Inputs=|++
  Sum1 : Sum  Inputs=|+-
  Sum2 : Sum  Inputs=|+-
  Sum3 : Sum  Inputs=|-+
  id : Outport
  iq : Outport  Port=2
  v_outd : Outport  Port=3
  v_outq : Outport  Port=4
  wires:
  v_in_q/1 -> Sum2/1  "v_in_q"
  v_in_d/1 -> Sum1/1  "v_in_d"
  v_out_q/1 -> v_outq/1, Sum2/2  "v_out_q"
  v_out_d/1 -> v_outd/1, Sum1/2  "v_out_d"
  Sum1/1 -> Gain/1  "vd"
  Sum2/1 -> Gain2/1  "vq"
  Gain/1 -> Gain5/1, Gain3/1
  Gain3/1 -> Sum/1
  Gain4/1 -> Sum/2
  Gain2/1 -> Gain6/1, Gain4/1
  Sum/1 -> id/1
  Gain5/1 -> Sum3/1
  Sum3/1 -> iq/1
  Gain6/1 -> Sum3/2

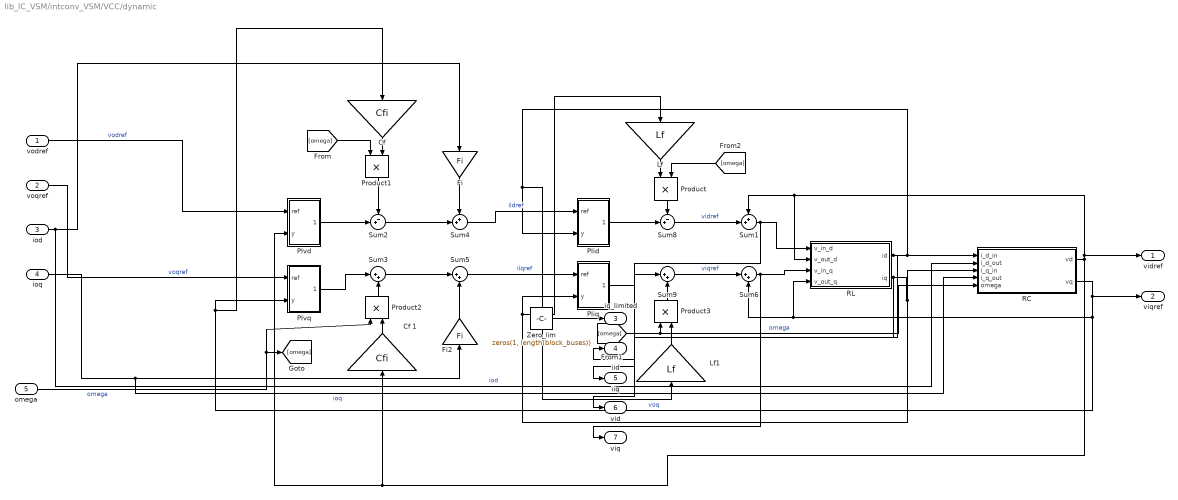
== system lib_IC_VSM/intconv_VSM/VCC/dynamic ==
  vodref : Inport
  voqref : Inport  Port=2
  iod : Inport  Port=3
  ioq : Inport  Port=4
  omega : Inport  Port=5
  Cf : Gain  Gain=Cfi
  Cf 1 : Gain  Gain=Cfi
  Fi : Gain  Gain=Fi
  Fi2 : Gain  Gain=Fi
  "Lf " : Gain  Gain=Lf
  Lf1 : Gain  Gain=Lf
  PIid : Subsystem
  PIiq : Subsystem
  PIvd : Subsystem
  PIvq : Subsystem
  Product{,1..3} (4 alike) : Product
  RC : Subsystem  Variant=on  mask{dynamic=Dynamic, R=Rcf, C=Cfi, fbase=50}
      mask prompts: dynamic "Dynamic behavior"; R "Parallel resistance (p.u.)"; C "Capacitance (p.u.)"; fbase "Base frequency (Hz)"
      mask init:
      | [iC, iR, omegab, rc_mode] = mask_init_RC(dynamic, R, C, fbase);
      mask TypeOptions dynamic: Dynamic | Static | Static omega
  RL : Subsystem  Variant=on  mask(Line){dynamic=Dynamic, R=Rf, L=Lf, fbase=fb}
      mask prompts: dynamic "Dynamic behavior"; R "Series resistance (p.u.)"; L "Inductance (p.u.)"; fbase "Base frequency (Hz)"
      mask init:
      | [invL, omegab, rl_mode] = mask_init_RL(dynamic, L, fbase);
      mask Help: web('Documentation/RL.html')
      mask TypeOptions dynamic: Static | Dynamic | Static omega
  Sum1 : Sum  Inputs=++|
  Sum2 : Sum  Inputs=-+|
  Sum{3,5..6,9} (4 alike) : Sum  Inputs=|++
  Sum4 : Sum  Inputs=++|
  Sum8 : Sum  Inputs=-+|
  Zero_lim : Constant  Value=zeros(1, length(block_buses))
  vidref : Outport
  viqref : Outport  Port=2
  iq_limited : Outport  Port=3
  iid : Outport  Port=4
  iiq : Outport  Port=5
  vid : Outport  Port=6
  viq : Outport  Port=7
  wires:
  Sum5/1 -> PIiq/1(ref)  "ilqref"
  Product/1 -> Sum8/1
  vodref/1 -> PIvd/1(ref)  "vodref"
  RC/2(vq) -> viqref/1, Sum6/2, RL/4(v_out_q), PIvq/2(y), Cf/1  "voq"
  [omega] -> Product/2
  Lf1/1 -> Product3/2
  Fi/1 -> Sum4/1
  voqref/1 -> PIvq/1(ref)  "voqref"
  Product3/1 -> Sum9/2
  Product2/1 -> Sum3/2
  Cf 1/1 -> Product2/2
  Cf/1 -> Product1/2
  Sum4/1 -> PIid/1(ref)  "ildref"
  Product1/1 -> Sum2/1
  iod/1 -> RC/2(i_d_out), Fi/1  "iod"
  Sum2/1 -> Sum4/2
  "Lf "/1 -> Product/1
  Sum3/1 -> Sum5/1
  [omega] -> RC/5(omega), Product3/1  "omega"
  ioq/1 -> RC/4(i_q_out), Fi2/1  "ioq"
  Fi2/1 -> Sum5/2
  PIvd/1(Out1) -> Sum2/2
  PIvq/1(Out1) -> Sum3/1
  PIid/1(Out1) -> Sum8/2
  PIiq/1(Out1) -> Sum9/1
  omega/1 -> Product2/1, [omega]  "omega"
  [omega] -> Product1/1
  RC/1(vd) -> vidref/1, Sum1/1, RL/2(v_out_d), PIvd/2(y), Cf 1/1
  RL/1(id) -> PIid/2(y), Lf1/1, RC/1(i_d_in), iid/1
  RL/2(iq) -> RC/3(i_q_in), PIiq/2(y), "Lf "/1, iiq/1
  Sum8/1 -> Sum1/2  "vidref"
  Sum9/1 -> Sum6/1  "viqref"
  Sum1/1 -> RL/1(v_in_d), vid/1
  Sum6/1 -> RL/3(v_in_q), viq/1
  Zero_lim/1 -> iq_limited/1

== system lib_IC_VSM/intconv_VSM/VCC/dynamic_VC ==
  vodref : Inport
  voqref : Inport  Port=2
  iod : Inport  Port=3
  ioq : Inport  Port=4
  omega : Inport  Port=5
  Cf : Gain  Gain=Cfi
  Cf 1 : Gain  Gain=Cfi
  Fi : Gain  Gain=Fi
  Fi2 : Gain  Gain=Fi
  Product1 : Product
  Product2 : Product
  RC : Subsystem  Variant=on  mask{dynamic=Dynamic, R=Rcf, C=Cfi, fbase=50}
      mask prompts: dynamic "Dynamic behavior"; R "Parallel resistance (p.u.)"; C "Capacitance (p.u.)"; fbase "Base frequency (Hz)"
      mask init:
      | [iC, iR, omegab, rc_mode] = mask_init_RC(dynamic, R, C, fbase);
      mask TypeOptions dynamic: Dynamic | Static | Static omega
  Subsystem : Subsystem
  Subsystem1 : Subsystem
  Sum2 : Sum  Inputs=-+|
  Sum3 : Sum  Inputs=|++
  Sum4 : Sum  Inputs=++|
  Sum5 : Sum  Inputs=|++
  vidref : Outport
  viqref : Outport  Port=2
  wires:
  [omega] -> Product1/1
  omega/1 -> RC/5(omega), Product2/1, [omega]  "omega"
  Subsystem1/1(Out1) -> Sum3/1
  Subsystem/1(Out1) -> Sum2/2
  Fi2/1 -> Sum5/2
  ioq/1 -> RC/4(i_q_out), Fi2/1  "ioq"
  Sum3/1 -> Sum5/1
  Sum2/1 -> Sum4/2
  iod/1 -> RC/2(i_d_out), Fi/1  "iod"
  Product1/1 -> Sum2/1
  Cf/1 -> Product1/2
  Cf 1/1 -> Product2/2
  Product2/1 -> Sum3/2
  voqref/1 -> Subsystem1/1(ref)  "voqref"
  Fi/1 -> Sum4/1
  RC/2(v_q) -> viqref/1, Cf/1, Subsystem1/2(y)
  vodref/1 -> Subsystem/1(ref)  "vodref"
  RC/1(v_d) -> vidref/1, Cf 1/1, Subsystem/2(y)
  Sum4/1 -> RC/1(i_d_in)
  Sum5/1 -> RC/3(i_q_in)

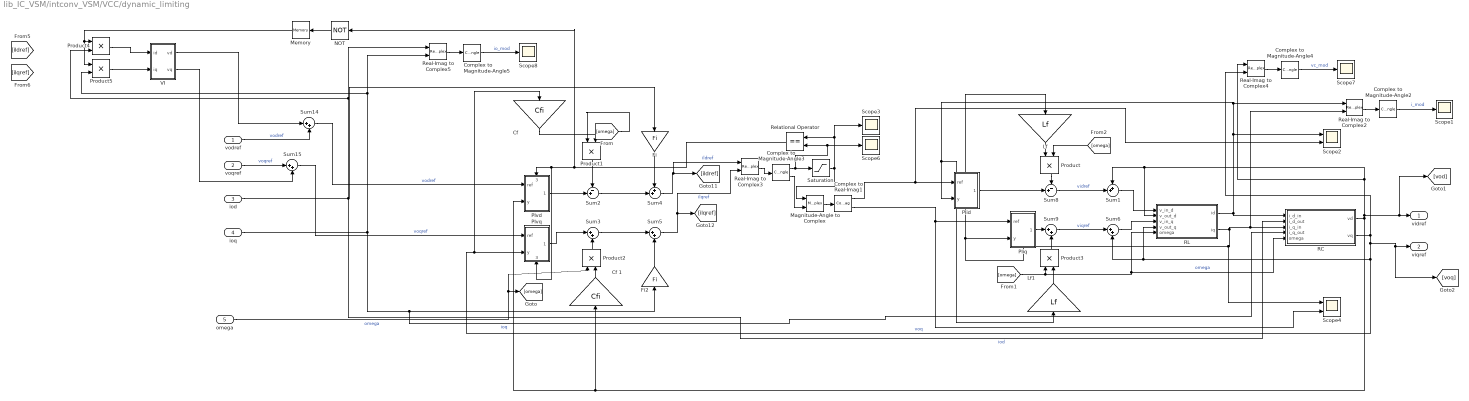
== system lib_IC_VSM/intconv_VSM/VCC/dynamic_limiting ==
  vodref : Inport
  voqref : Inport  Port=2
  iod : Inport  Port=3
  ioq : Inport  Port=4
  omega : Inport  Port=5
  Cf : Gain  Gain=Cfi
  Cf 1 : Gain  Gain=Cfi
  Complex to Magnitude-Angle2 : ComplexToMagnitudeAngle  Output=Magnitude
  Complex to Magnitude-Angle3 : ComplexToMagnitudeAngle
  Complex to Magnitude-Angle4 : ComplexToMagnitudeAngle  Output=Magnitude
  Complex to Magnitude-Angle5 : ComplexToMagnitudeAngle  Output=Magnitude
  Complex to Real-Imag1 : ComplexToRealImag
  Fi : Gain  Gain=Fi
  Fi2 : Gain  Gain=Fi
  "Lf " : Gain  Gain=Lf
  Lf1 : Gain  Gain=Lf
  Magnitude-Angle to Complex : MagnitudeAngleToComplex
  Memory : Memory
  NOT : Logic  Operator=NOT  IconShape=distinctive  AllPortsSameDT=off  OutDataTypeStr=boolean
  PIid : Subsystem
  PIiq : Subsystem
  PIvd : Subsystem
      settings: PortSchema="{\"entries\":[{\"content\":{\"sides\":[{\"content\":{\"connectorIds\":[\"In1\",\"In2\"]},\"type\":\"ConnectorPlacement.EquallySpacedRectSide\",\"uuid\":\"218efe14-094c-4cdd-8e62-ef6089c75bbd\"},{\"content\":{\"connectorIds\":[\"Out1\"],\"side\":\"RIGHT\"},\"type\":\"ConnectorPlacement.EquallySpacedRectSide\",\"uuid\":\"287e2a8a-062a-4519-a86c-f141c6982dac\"},{\"content\":{\"connectorIds\":[\"In3\"],\"side\":\"TOP\"},\"type\":\"ConnectorPlacement.EquallySpacedRectSide\",\"uuid\":\"e88fce21-908c-492a-b265-04b05ce94be8\"}]},\"type\":\"ConnectorPlacement.EquallySpacedConnector\",\"uuid\":\"5c149457-da6d-4223-b1cb-56365173b759\"}],\"packageUris\":[\"http://schema.mathworks.com/mf0/Connector/R2020b\"],\"version\":\"1.0\"}"
  PIvq : Subsystem
      settings: PortSchema="{\"entries\":[{\"content\":{\"sides\":[{\"content\":{\"connectorIds\":[\"In1\",\"In2\"]},\"type\":\"ConnectorPlacement.EquallySpacedRectSide\",\"uuid\":\"218efe14-094c-4cdd-8e62-ef6089c75bbd\"},{\"content\":{\"connectorIds\":[\"Out1\"],\"side\":\"RIGHT\"},\"type\":\"ConnectorPlacement.EquallySpacedRectSide\",\"uuid\":\"287e2a8a-062a-4519-a86c-f141c6982dac\"},{\"content\":{\"connectorIds\":[],\"side\":\"TOP\"},\"type\":\"ConnectorPlacement.EquallySpacedRectSide\",\"uuid\":\"e88fce21-908c-492a-b265-04b05ce94be8\"},{\"content\":{\"connectorIds\":[\"In3\"],\"side\":\"BOTTOM\"},\"type\":\"ConnectorPlacement.EquallySpacedRectSide\",\"uuid\":\"db964aea-37c6-4226-90b6-d177a6d2ab38\"}]},\"type\":\"ConnectorPlacement.EquallySpacedConnector\",\"uuid\":\"5c149457-da6d-4223-b1cb-56365173b759\"}],\"packageUris\":[\"http://schema.mathworks.com/mf0/Connector/R2020b\"],\"version\":\"1.0\"}"
  Product{,1..5} (6 alike) : Product
  RC : Subsystem  Variant=on  mask{dynamic=Dynamic, R=Rcf, C=Cfi}
      mask prompts: dynamic "Dynamic behavior"; R "Parallel resistance (p.u.)"; C "Capacitance (p.u.)"
      mask init:
      | [iC, iR, omegab, rc_mode] = mask_init_RC(dynamic, R, C, 50);
      mask TypeOptions dynamic: Dynamic | Static | Static omega
  RL : Subsystem  Variant=on  mask(Line){dynamic=Dynamic, R=Rf, L=Lf}
      mask prompts: dynamic "Dynamic behavior"; R "Series resistance (p.u.)"; L "Inductance (p.u.)"
      mask init:
      | [invL, omegab, rl_mode] = mask_init_RL(dynamic, L, 50);
      mask Help: web('Documentation/RL.html')
      mask TypeOptions dynamic: Static | Dynamic | Static omega
  Real-Imag to Complex{2..5} (4 alike) : RealImagToComplex
  Relational Operator : RelationalOperator  Operator===  OutDataTypeStr=boolean  RndMeth=Simplest  InputSameDT=off
  Saturation : Saturate  UpperLimit=0.1  LowerLimit=0
  Scope{1,3,6..8} (5 alike) : Scope
      Scope1 settings: ActiveDisplayYMinimum=-0.06728  ActiveDisplayYMaximum=0.79818  DataLoggingVariableName=ScopeData2
      Scope3 settings: ActiveDisplayYMinimum=0.01769  ActiveDisplayYMaximum=0.10915
      Scope6 settings: ActiveDisplayYMinimum=0.03196  ActiveDisplayYMaximum=0.13112  DataLoggingVariableName=ScopeData2
      Scope7 settings: ActiveDisplayYMinimum=0.86043  ActiveDisplayYMaximum=1.1554  DataLoggingVariableName=ScopeData3
      Scope8 settings: ActiveDisplayYMinimum=0.0318  ActiveDisplayYMaximum=0.12782  DataLoggingVariableName=ScopeData4
  Scope2 : Scope  NumInputPorts=2
      settings: ActiveDisplayYMinimum=-0.10019  ActiveDisplayYMaximum=0.20176
  Scope4 : Scope  NumInputPorts=2
      settings: ActiveDisplayYMinimum=-0.04364  ActiveDisplayYMaximum=0.0791  DataLoggingVariableName=ScopeData3
  Sum1 : Sum  Inputs=++|
  Sum{3,5..6,9,14..15} (6 alike) : Sum  Inputs=|++
  Sum2 : Sum  Inputs=-+|
  Sum4 : Sum  Inputs=++|
  Sum8 : Sum  Inputs=-+|
  VI : Subsystem  mask{L=0.5, R=0.1, Tf=0}
      mask prompts: L "Inductance (pu)"; R "Resistance (pu)"; Tf "WOF time constant (s)"
      mask init:
      | [iTf, use_Tf] = mask_init_opt_filter(Tf);
  vidref : Outport
  viqref : Outport  Port=2
  wires:
  Product/1 -> Sum8/1
  Sum14/1 -> PIvd/1(ref)  "vodref"
  RC/2(vq) -> [voq], viqref/1, RL/4(v_out_q), Sum6/2, PIvq/2(y), Cf/1, Real-Imag to Complex4/2  "voq"
  [omega] -> Product/2
  Lf1/1 -> Product3/2
  Fi/1 -> Sum4/1
  Sum15/1 -> PIvq/1(ref)  "voqref"
  Product3/1 -> Sum9/2
  Product2/1 -> Sum3/2
  Cf 1/1 -> Product2/2
  Cf/1 -> Product1/2
  Product1/1 -> Sum2/1
  iod/1 -> RC/2(i_d_out), Real-Imag to Complex5/1, Product4/2, Fi/1  "iod"
  Sum2/1 -> Sum4/2
  "Lf "/1 -> Product/1
  Sum3/1 -> Sum5/1
  [omega] -> RC/5(omega), RL/5(omega), Product3/1  "omega"
  ioq/1 -> RC/4(i_q_out), Fi2/1, Real-Imag to Complex5/2, Product5/2  "ioq"
  Fi2/1 -> Sum5/2
  PIvd/1(Out1) -> Sum2/2
  PIvq/1(Out1) -> Sum3/1
  PIid/1(Out1) -> Sum8/2
  PIiq/1(Out1) -> Sum9/1
  omega/1 -> Product2/1, [omega]  "omega"
  [omega] -> Product1/1
  RL/1(id) -> RC/1(i_d_in), Scope2/1, Real-Imag to Complex2/1, PIid/2(y), Lf1/1
  RL/2(iq) -> Scope4/1, PIiq/2(y), "Lf "/1, Real-Imag to Complex2/2, RC/3(i_q_in)
  Sum8/1 -> Sum1/2  "vidref"
  Sum9/1 -> Sum6/1  "viqref"
  Sum1/1 -> RL/1(v_in_d)
  Sum6/1 -> RL/3(v_in_q)
  Sum4/1 -> Real-Imag to Complex3/1, [ildref]  "ildref"
  Sum5/1 -> Real-Imag to Complex3/2, [ilqref]  "ilqref"
  RC/1(vd) -> Real-Imag to Complex4/1, RL/2(v_out_d), Sum1/1, [vod], vidref/1, PIvd/2(y), Cf 1/1
  Complex to Real-Imag1/2 -> Scope4/2, PIiq/1(ref)
  Real-Imag to Complex2/1 -> Complex to Magnitude-Angle2/1
  Complex to Magnitude-Angle2/1 -> Scope1/1  "i_mod"
  Complex to Real-Imag1/1 -> Scope2/2, PIid/1(ref)
  Real-Imag to Complex3/1 -> Complex to Magnitude-Angle3/1
  Saturation/1 -> Magnitude-Angle to Complex/1, Scope3/1, Relational Operator/1
  Relational Operator/1 -> PIvd/3(anti_windup), PIvq/3(anti_windup), NOT/1
  Complex to Magnitude-Angle3/1 -> Scope6/1, Relational Operator/2, Saturation/1
  Magnitude-Angle to Complex/1 -> Complex to Real-Imag1/1
  Complex to Magnitude-Angle3/2 -> Magnitude-Angle to Complex/2
  Complex to Magnitude-Angle4/1 -> Scope7/1  "vc_mod"
  Real-Imag to Complex4/1 -> Complex to Magnitude-Angle4/1
  Real-Imag to Complex5/1 -> Complex to Magnitude-Angle5/1
  Complex to Magnitude-Angle5/1 -> Scope8/1  "io_mod"
  vodref/1 -> Sum14/2  "vodref"
  voqref/1 -> Sum15/1  "voqref"
  NOT/1 -> Memory/1
  VI/1(vd) -> Sum14/1
  VI/2(vq) -> Sum15/2
  Memory/1 -> Product5/1, Product4/1
  Product4/1 -> VI/1(id)
  Product5/1 -> VI/2(iq)

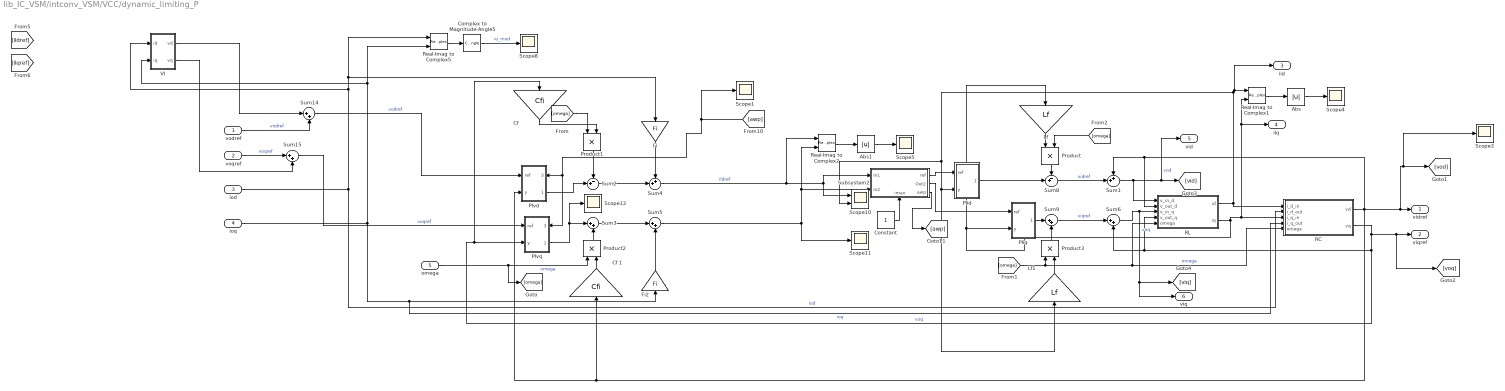
== system lib_IC_VSM/intconv_VSM/VCC/dynamic_limiting_P ==
  vodref : Inport
  voqref : Inport  Port=2
  iod : Inport  Port=3
  ioq : Inport  Port=4
  omega : Inport  Port=5
  Abs : Abs  SaturateOnIntegerOverflow=off
  Abs1 : Abs  SaturateOnIntegerOverflow=off
  Cf : Gain  Gain=Cfi
  Cf 1 : Gain  Gain=Cfi
  Complex to Magnitude-Angle5 : ComplexToMagnitudeAngle  Output=Magnitude
  Constant : Constant
  Fi : Gain  Gain=Fi
  Fi2 : Gain  Gain=Fi
  "Lf " : Gain  Gain=Lf
  Lf1 : Gain  Gain=Lf
  PIid : Subsystem
  PIiq : Subsystem
  PIvd : Subsystem
      settings: PortSchema="{\"entries\":[{\"content\":{\"sides\":[{\"content\":{\"connectorIds\":[\"In1\",\"In2\"]},\"type\":\"ConnectorPlacement.EquallySpacedRectSide\",\"uuid\":\"218efe14-094c-4cdd-8e62-ef6089c75bbd\"},{\"content\":{\"connectorIds\":[\"In3\",\"Out1\"],\"side\":\"RIGHT\"},\"type\":\"ConnectorPlacement.EquallySpacedRectSide\",\"uuid\":\"287e2a8a-062a-4519-a86c-f141c6982dac\"},{\"content\":{\"side\":\"TOP\"},\"type\":\"ConnectorPlacement.EquallySpacedRectSide\",\"uuid\":\"e88fce21-908c-492a-b265-04b05ce94be8\"}]},\"type\":\"ConnectorPlacement.EquallySpacedConnector\",\"uuid\":\"5c149457-da6d-4223-b1cb-56365173b759\"}],\"packageUris\":[\"http://schema.mathworks.com/mf0/Connector/R2020b\"],\"version\":\"1.0\"}"
  PIvq : Subsystem
      settings: PortSchema="{\"entries\":[{\"content\":{\"sides\":[{\"content\":{\"connectorIds\":[\"In1\",\"In2\"]},\"type\":\"ConnectorPlacement.EquallySpacedRectSide\",\"uuid\":\"5bfd4306-8421-4fdd-bae9-79740558d514\"},{\"content\":{\"connectorIds\":[\"In3\",\"Out1\"],\"side\":\"RIGHT\"},\"type\":\"ConnectorPlacement.EquallySpacedRectSide\",\"uuid\":\"1419fa8e-cc02-4da2-9592-d06db5fac946\"},{\"content\":{\"side\":\"TOP\"},\"type\":\"ConnectorPlacement.EquallySpacedRectSide\",\"uuid\":\"32aa87b6-be70-473d-807b-ed4692b27e5a\"}]},\"type\":\"ConnectorPlacement.EquallySpacedConnector\",\"uuid\":\"6bf6a9bf-c4c4-4ccc-a31e-1b4c70dd37d4\"}],\"packageUris\":[\"http://schema.mathworks.com/mf0/Connector/R2020b\"],\"version\":\"1.0\"}"
  Product{,1..3} (4 alike) : Product
  RC : Subsystem  Variant=on  mask{dynamic=Dynamic, R=Rcf, C=Cfi}
      mask prompts: dynamic "Dynamic behavior"; R "Parallel resistance (p.u.)"; C "Capacitance (p.u.)"
      mask init:
      | [iC, iR, omegab, rc_mode] = mask_init_RC(dynamic, R, C, 50);
      mask TypeOptions dynamic: Dynamic | Static | Static omega
  RL : Subsystem  Variant=on  mask(Line){dynamic=Dynamic, R=Rf, L=Lf}
      mask prompts: dynamic "Dynamic behavior"; R "Series resistance (p.u.)"; L "Inductance (p.u.)"
      mask init:
      | [invL, omegab, rl_mode] = mask_init_RL(dynamic, L, 50);
      mask Help: web('Documentation/RL.html')
      mask TypeOptions dynamic: Static | Dynamic | Static omega
  Real-Imag to Complex1 : RealImagToComplex
  Real-Imag to Complex2 : RealImagToComplex
  Real-Imag to Complex5 : RealImagToComplex
  Scope{1,3..5,8,11..12} (7 alike) : Scope
      Scope1 settings: ActiveDisplayYMinimum=-0.125  ActiveDisplayYMaximum=1.125  DataLoggingVariableName=ScopeData2
      Scope11 settings: ActiveDisplayYMinimum=-166.4137  ActiveDisplayYMaximum=84.6213  DataLoggingVariableName=ScopeData2
      Scope12 settings: ActiveDisplayYMinimum=-1  ActiveDisplayYMaximum=1  DataLoggingVariableName=ScopeData3
      Scope3 settings: ActiveDisplayYMinimum=0.77192  ActiveDisplayYMaximum=1.1413  DataLoggingVariableName=ScopeData4
      Scope4 settings: ActiveDisplayYMinimum=0.18699  ActiveDisplayYMaximum=0.31058  DataLoggingVariableName=ScopeData6
      Scope5 settings: ActiveDisplayYMinimum=-1  ActiveDisplayYMaximum=1
      Scope8 settings: ActiveDisplayYMinimum=-1  ActiveDisplayYMaximum=1  DataLoggingVariableName=ScopeData4
  Scope10 : Scope  NumInputPorts=2
      settings: ActiveDisplayYMinimum=0.12846  ActiveDisplayYMaximum=0.33105
  Subsystem2 : Subsystem
      settings: PortSchema="{\"entries\":[{\"content\":{\"sides\":[{\"content\":{\"connectorIds\":[\"In1\",\"In2\"]},\"type\":\"ConnectorPlacement.EquallySpacedRectSide\",\"uuid\":\"9ad25d09-f130-47a3-8a0c-c3d50f40a3f5\"},{\"content\":{\"connectorIds\":[\"Out1\",\"Out2\",\"Out3\"],\"side\":\"RIGHT\"},\"type\":\"ConnectorPlacement.EquallySpacedRectSide\",\"uuid\":\"00c4c943-52e8-4170-9ba5-4d3b10561d7b\"},{\"content\":{\"side\":\"TOP\"},\"type\":\"ConnectorPlacement.EquallySpacedRectSide\",\"uuid\":\"98a959d8-b430-483b-8e6f-0eab01c1bae1\"},{\"content\":{\"connectorIds\":[\"In3\"],\"side\":\"BOTTOM\"},\"type\":\"ConnectorPlacement.EquallySpacedRectSide\",\"uuid\":\"01418333-d465-4764-adcc-2e5b92b6bf5d\"}]},\"type\":\"ConnectorPlacement.EquallySpacedConnector\",\"uuid\":\"e741d9d4-93b5-4bd9-8695-3e699c12860d\"}],\"packageUris\":[\"http://schema.mathworks.com/mf0/Connector/R2020b\"],\"version\":\"1.0\"}"
  Sum1 : Sum  Inputs=++|
  Sum{3,5..6,9,14..15} (6 alike) : Sum  Inputs=|++
  Sum2 : Sum  Inputs=-+|
  Sum4 : Sum  Inputs=++|
  Sum8 : Sum  Inputs=-+|
  VI : Subsystem  mask{L=0, R=0, Tf=0}
      mask prompts: L "Inductance (pu)"; R "Resistance (pu)"; Tf "WOF time constant (s)"
      mask init:
      | [iTf, use_Tf] = mask_init_opt_filter(Tf);
  vidref : Outport
  viqref : Outport  Port=2
  iid : Outport  Port=3
  iiq : Outport  Port=4
  vid : Outport  Port=5
  viq : Outport  Port=6
  wires:
  Product/1 -> Sum8/1
  Sum14/1 -> PIvd/1(ref)  "vodref"
  RC/2(vq) -> [voq], viqref/1, RL/4(v_out_q), Sum6/2, PIvq/2(y), Cf/1  "voq"
  [omega] -> Product/2
  Lf1/1 -> Product3/2
  Sum15/1 -> PIvq/1(ref)  "voqref"
  Product3/1 -> Sum9/2
  Cf 1/1 -> Product2/2
  Cf/1 -> Product1/2
  Product1/1 -> Sum2/1
  iod/1 -> VI/1(id), Fi/1, Real-Imag to Complex5/1, RC/2(i_d_out)  "iod"
  Sum2/1 -> Sum4/2
  "Lf "/1 -> Product/1
  Sum3/1 -> Sum5/1
  [omega] -> RL/5(omega), RC/5(omega), Product3/1  "omega"
  ioq/1 -> RC/4(i_q_out), Fi2/1, VI/2(iq), Real-Imag to Complex5/2  "ioq"
  PIvd/1(Out1) -> Sum2/2
  PIvq/1(Out1) -> Scope12/1, Sum3/1
  PIid/1(Out1) -> Sum8/2
  PIiq/1(Out1) -> Sum9/1
  omega/1 -> [omega], Product2/1  "omega"
  [omega] -> Product1/1
  RL/1(id) -> RC/1(i_d_in), iid/1, Real-Imag to Complex1/1, PIid/2(y), Lf1/1, Scope10/2
  RL/2(iq) -> PIiq/2(y), "Lf "/1, iiq/1, Real-Imag to Complex1/2, RC/3(i_q_in)
  Sum8/1 -> Sum1/2  "vidref"
  Sum9/1 -> Sum6/1  "viqref"
  RC/1(vd) -> RL/2(v_out_d), Sum1/1, Scope3/1, [vod], vidref/1, PIvd/2(y), Cf 1/1
  Real-Imag to Complex5/1 -> Complex to Magnitude-Angle5/1
  Complex to Magnitude-Angle5/1 -> Scope8/1  "io_mod"
  vodref/1 -> Sum14/2  "vodref"
  voqref/1 -> Sum15/1  "voqref"
  VI/1(vd) -> Sum14/1
  VI/2(vq) -> Sum15/2
  Sum6/1 -> viq/1, [viq], RL/3(v_in_q)  "voq"
  Sum1/1 -> RL/1(v_in_d), vid/1, [vid]  "vod"
  Abs/1 -> Scope4/1
  Real-Imag to Complex1/1 -> Abs/1
  Sum5/1 -> Subsystem2/2(In2), Real-Imag to Complex2/2, Scope11/1
  Real-Imag to Complex2/1 -> Abs1/1
  Abs1/1 -> Scope5/1
  Fi/1 -> Sum4/1
  [awp] -> PIvd/3(awp), PIvq/3(awp), Scope1/1
  Product2/1 -> Sum3/2
  Fi2/1 -> Sum5/2
  Subsystem2/1(ref) -> PIid/1(ref)
  Subsystem2/2(Out2) -> PIiq/1(ref)
  Constant/1 -> Subsystem2/3(imax)
  Subsystem2/3(awp) -> [awp]
  Sum4/1 -> Real-Imag to Complex2/1, Subsystem2/1(In1), Scope10/1  "ildref"

== system lib_IC_VSM/intconv_VSM/VCC/static ==
  vodref : Inport
  voqref : Inport  Port=2
  iod : Inport  Port=3
  ioq : Inport  Port=4
  omega : Inport  Port=5
  Terminator : Terminator
  Terminator1 : Terminator
  Terminator2 : Terminator
  Zero_lim : Constant  Value=zeros(1, length(block_buses))
  vidref : Outport
  viqref : Outport  Port=2
  iq_limited : Outport  Port=3
  iid : Outport  Port=4
  iiq : Outport  Port=5
  vid : Outport  Port=6
  viq : Outport  Port=7
  wires:
  voqref/1 -> viqref/1, viq/1  "voqref"
  vodref/1 -> vidref/1, vid/1  "vodref"
  iod/1 -> Terminator/1, iid/1  "iod"
  ioq/1 -> Terminator1/1, iiq/1  "ioq"
  omega/1 -> Terminator2/1  "ioq"
  Zero_lim/1 -> iq_limited/1

== system lib_IC_VSM/intconv_VSM/VI/WOF_d ==
  note: 1) Add Subsystem or Model blocks as valid variant choices.
      | 2) You cannot connect blocks at this level. At simulation, connectivity is automatically
      | determined, based on the active variant and port name matching.
  In1 : Inport
  Active : Subsystem  VariantControl=use_Tf == 1
  Bypass : Subsystem  VariantControl=(default)
  Out1 : Outport
